simulink model "fw_io_out_hw"  (R2026b)
settings: Solver=VariableStepAuto
undefined symbols (not defined in the file or in its folder): CAN, FD, P, Ts
libraries: stm32blockslib x8, stm32f4xxblockslib x4, simulink x1, stmutilitieslib x1
settings Model: Creator=aomar  LastModifiedBy=aomar

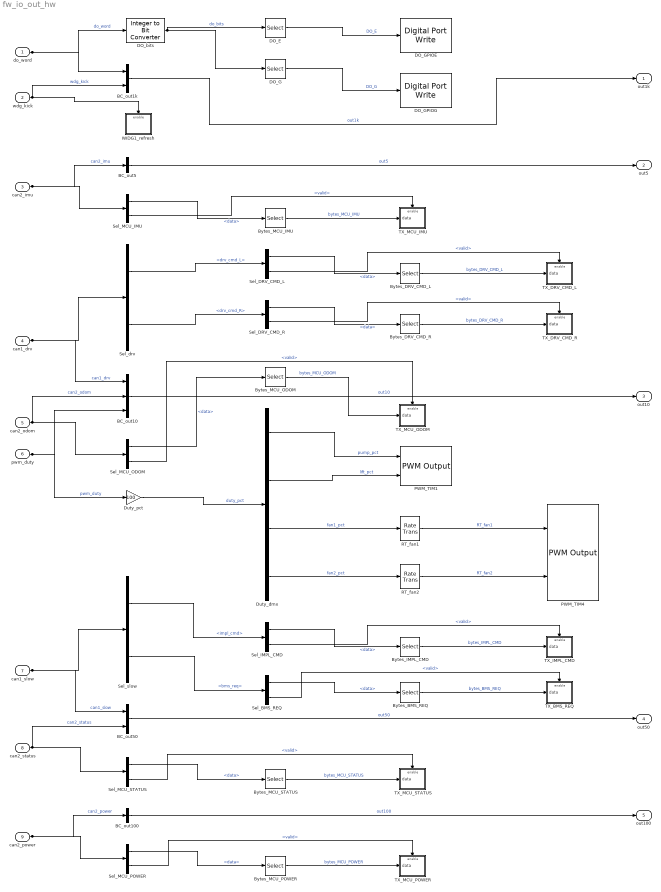
== system fw_io_out_hw ==
  do_word : Inport  OutDataTypeStr=uint32  SampleTime=Ts.base
  wdg_kick : Inport  Port=2  OutDataTypeStr=boolean  SampleTime=Ts.base
  can2_imu : Inport  Port=3  OutDataTypeStr=Bus: Bus_CanFrame64  SampleTime=Ts.imu
  can1_drv : Inport  Port=4  OutDataTypeStr=Bus: Bus_Can1_McuFast  SampleTime=Ts.ctrl
  can2_odom : Inport  Port=5  OutDataTypeStr=Bus: Bus_CanFrame64  SampleTime=Ts.ctrl
  pwm_duty : Inport  Port=6  OutDataTypeStr=single  PortDimensions=4  SampleTime=Ts.ctrl
  can1_slow : Inport  Port=7  OutDataTypeStr=Bus: Bus_Can1_McuSlow  SampleTime=Ts.comm
  can2_status : Inport  Port=8  OutDataTypeStr=Bus: Bus_CanFrame64  SampleTime=Ts.comm
  can2_power : Inport  Port=9  OutDataTypeStr=Bus: Bus_CanFrame64  SampleTime=Ts.hk
  BC_out10 : BusCreator  Inputs=3  OutDataTypeStr=Bus: Bus_McuOut10  NonVirtualBus=on
      settings: InheritFromInputs=off
  BC_out100 : BusCreator  Inputs=1  OutDataTypeStr=Bus: Bus_McuOut100  NonVirtualBus=on
      settings: InheritFromInputs=off
  BC_out1k : BusCreator  Inputs=2  OutDataTypeStr=Bus: Bus_McuOut1k  NonVirtualBus=on
      settings: InheritFromInputs=off
  BC_out5 : BusCreator  Inputs=1  OutDataTypeStr=Bus: Bus_McuOut5  NonVirtualBus=on
      settings: InheritFromInputs=off
  BC_out50 : BusCreator  Inputs=2  OutDataTypeStr=Bus: Bus_McuOut50  NonVirtualBus=on
      settings: InheritFromInputs=off
  Bytes_BMS_REQ : Selector  InputPortWidth=8  IndexOptions=Index vector (dialog)  Indices=1:8  OutputSizes=1
  Bytes_DRV_CMD_L : Selector  InputPortWidth=8  IndexOptions=Index vector (dialog)  Indices=1:8  OutputSizes=1
  Bytes_DRV_CMD_R : Selector  InputPortWidth=8  IndexOptions=Index vector (dialog)  Indices=1:8  OutputSizes=1
  Bytes_IMPL_CMD : Selector  InputPortWidth=8  IndexOptions=Index vector (dialog)  Indices=1:8  OutputSizes=1
  Bytes_MCU_IMU : Selector  InputPortWidth=64  IndexOptions=Index vector (dialog)  Indices=1:48  OutputSizes=1
  Bytes_MCU_ODOM : Selector  InputPortWidth=64  IndexOptions=Index vector (dialog)  Indices=1:32  OutputSizes=1
  Bytes_MCU_POWER : Selector  InputPortWidth=64  IndexOptions=Index vector (dialog)  Indices=1:64  OutputSizes=1
  Bytes_MCU_STATUS : Selector  InputPortWidth=64  IndexOptions=Index vector (dialog)  Indices=1:48  OutputSizes=1
  DO_E : Selector  InputPortWidth=32  IndexOptions=Index vector (dialog)  Indices=P.electronics.hw.do_g_pins+(1:P.electronics.hw.do_e_pins)  OutputSizes=1
  DO_G : Selector  InputPortWidth=32  IndexOptions=Index vector (dialog)  Indices=1:P.electronics.hw.do_g_pins  OutputSizes=1
  DO_GPIOE : stm32f4xxblockslib/Digital Port Write  PortName=GPIOE  PinNumber=[0:3]  ReadOperation=off  IOAsArray=on  EnableSimPort=off  hoistedMaskSrc=ECSoC/ECSimCodegen/Digital Port Write
      settings: LibrarySourceBlock=stm32h7xxblockslib/Digital Port Write
  DO_GPIOG : stm32f4xxblockslib/Digital Port Write  PortName=GPIOG  PinNumber=[0:15]  ReadOperation=off  IOAsArray=on  EnableSimPort=off  hoistedMaskSrc=ECSoC/ECSimCodegen/Digital Port Write
      settings: LibrarySourceBlock=stm32h7xxblockslib/Digital Port Write
  DO_bits : simulink/Logic and Bit Operations/Integer to Bit Converter  nbits=32  signedInputValues=Unsigned  bitOrder=LSB first  outDtype=boolean
      settings: LibrarySourceBlock=|
      | commutil2/Integer to Bit
      | Converter
  Duty_dmx : Demux
  Duty_pct : Gain  Gain=100
  IWDG1_refresh : Subsystem
  PWM_TIM1 : stm32f4xxblockslib/PWM Output  ProcessorFamily=STM32G4  TimerModule=TIM1  DutycycleUnits=Percentage  EnableChannel1=on  EnableCaptureCompare1Input=off  EnableCaptureCompare1ComplementaryInput=off  EnableOutputCompare1ModeInput=off  EnableChannel2=on  EnableCaptureCompare2Input=off  EnableCaptureCompare2ComplementaryInput=off  EnableOutputCompare2ModeInput=off  EnableChannel3=off  EnableCaptureCompare3Input=off  EnableCaptureCompare3ComplementaryInput=off  EnableOutputCompare3ModeInput=off  EnableChannel4=off  EnableCaptureCompare4Input=off  EnableCaptureCompare4ComplementaryInput=off  EnableOutputCompare4ModeInput=off  EnableChannel5=off  EnableCaptureCompare5Input=off  EnableOutputCompare5ModeInput=off  EnableChannel6=off  EnableCaptureCompare6Input=off  EnableOutputCompare6ModeInput=off  EnableCounterInput=off  EnableMainOutputInput=off  EnableFrequencyInput=off  SetRCAfterCE=off  OutputDirection=off  OutputMainOutputEnableStatus=off  SampleTime=Ts.ctrl  EnableSimPort=off  EnableUpdateEvent=off  EnableCaptureCompare1Event=off  EnableCaptureCompare2Event=off  EnableCaptureCompare3Event=off  EnableCaptureCompare4Event=off  EnableTriggerEvent=off  EnableBreakEvent=off  EnableBreakEvent2=off  hoistedMaskSrc=ECSoC/ECSimCodegen/PWM Output
      settings: LibrarySourceBlock=stm32h7xxblockslib/PWM Output
  PWM_TIM4 : stm32f4xxblockslib/PWM Output  ProcessorFamily=STM32G4  TimerModule=TIM4  DutycycleUnits=Percentage  EnableChannel1=on  EnableCaptureCompare1Input=off  EnableCaptureCompare1ComplementaryInput=off  EnableOutputCompare1ModeInput=off  EnableChannel2=on  EnableCaptureCompare2Input=off  EnableCaptureCompare2ComplementaryInput=off  EnableOutputCompare2ModeInput=off  EnableChannel3=off  EnableCaptureCompare3Input=off  EnableCaptureCompare3ComplementaryInput=off  EnableOutputCompare3ModeInput=off  EnableChannel4=off  EnableCaptureCompare4Input=off  EnableCaptureCompare4ComplementaryInput=off  EnableOutputCompare4ModeInput=off  EnableChannel5=off  EnableCaptureCompare5Input=off  EnableOutputCompare5ModeInput=off  EnableChannel6=off  EnableCaptureCompare6Input=off  EnableOutputCompare6ModeInput=off  EnableCounterInput=off  EnableMainOutputInput=off  EnableFrequencyInput=off  SetRCAfterCE=off  OutputDirection=off  OutputMainOutputEnableStatus=off  SampleTime=Ts.hk  EnableSimPort=off  EnableUpdateEvent=off  EnableCaptureCompare1Event=off  EnableCaptureCompare2Event=off  EnableCaptureCompare3Event=off  EnableCaptureCompare4Event=off  EnableTriggerEvent=off  EnableBreakEvent=off  EnableBreakEvent2=off  hoistedMaskSrc=ECSoC/ECSimCodegen/PWM Output
      settings: LibrarySourceBlock=stm32h7xxblockslib/PWM Output
  RT_fan1 : RateTransition  OutPortSampleTime=Ts.hk
  RT_fan2 : RateTransition  OutPortSampleTime=Ts.hk
  Sel_BMS_REQ : BusSelector  OutputSignals=data,valid
  Sel_DRV_CMD_L : BusSelector  OutputSignals=data,valid
  Sel_DRV_CMD_R : BusSelector  OutputSignals=data,valid
  Sel_IMPL_CMD : BusSelector  OutputSignals=data,valid
  Sel_MCU_IMU : BusSelector  OutputSignals=data,valid
  Sel_MCU_ODOM : BusSelector  OutputSignals=data,valid
  Sel_MCU_POWER : BusSelector  OutputSignals=data,valid
  Sel_MCU_STATUS : BusSelector  OutputSignals=data,valid
  Sel_drv : BusSelector  OutputSignals=drv_cmd_L,drv_cmd_R
  Sel_slow : BusSelector  OutputSignals=impl_cmd,bms_req
  TX_BMS_REQ : Subsystem
  TX_DRV_CMD_L : Subsystem
  TX_DRV_CMD_R : Subsystem
  TX_IMPL_CMD : Subsystem
  TX_MCU_IMU : Subsystem
  TX_MCU_ODOM : Subsystem
  TX_MCU_POWER : Subsystem
  TX_MCU_STATUS : Subsystem
  out1k : Outport  OutDataTypeStr=Bus: Bus_McuOut1k
  out5 : Outport  Port=2  OutDataTypeStr=Bus: Bus_McuOut5
  out10 : Outport  Port=3  OutDataTypeStr=Bus: Bus_McuOut10
  out50 : Outport  Port=4  OutDataTypeStr=Bus: Bus_McuOut50
  out100 : Outport  Port=5  OutDataTypeStr=Bus: Bus_McuOut100
  wires:
  do_word/1 -> DO_bits/1, BC_out1k/1  "do_word"
  wdg_kick/1 -> IWDG1_refresh/Enable, BC_out1k/2  "wdg_kick"
  can2_imu/1 -> BC_out5/1, Sel_MCU_IMU/1  "can2_imu"
  can1_drv/1 -> Sel_drv/1, BC_out10/1  "can1_drv"
  can2_odom/1 -> Sel_MCU_ODOM/1, BC_out10/2  "can2_odom"
  pwm_duty/1 -> BC_out10/3, Duty_pct/1  "pwm_duty"
  can1_slow/1 -> Sel_slow/1, BC_out50/1  "can1_slow"
  can2_status/1 -> Sel_MCU_STATUS/1, BC_out50/2  "can2_status"
  can2_power/1 -> BC_out100/1, Sel_MCU_POWER/1  "can2_power"
  BC_out1k/1 -> out1k/1  "out1k"
  BC_out5/1 -> out5/1  "out5"
  Sel_MCU_IMU/1 -> Bytes_MCU_IMU/1  "<data>"
  Sel_MCU_IMU/2 -> TX_MCU_IMU/Enable  "<valid>"
  Sel_drv/1 -> Sel_DRV_CMD_L/1  "<drv_cmd_L>"
  Sel_drv/2 -> Sel_DRV_CMD_R/1  "<drv_cmd_R>"
  BC_out10/1 -> out10/1  "out10"
  Sel_MCU_ODOM/1 -> Bytes_MCU_ODOM/1  "<data>"
  Sel_MCU_ODOM/2 -> TX_MCU_ODOM/Enable  "<valid>"
  Sel_slow/1 -> Sel_IMPL_CMD/1  "<impl_cmd>"
  Sel_slow/2 -> Sel_BMS_REQ/1  "<bms_req>"
  BC_out50/1 -> out50/1  "out50"
  Sel_MCU_STATUS/1 -> Bytes_MCU_STATUS/1  "<data>"
  Sel_MCU_STATUS/2 -> TX_MCU_STATUS/Enable  "<valid>"
  BC_out100/1 -> out100/1  "out100"
  Sel_MCU_POWER/1 -> Bytes_MCU_POWER/1  "<data>"
  Sel_MCU_POWER/2 -> TX_MCU_POWER/Enable  "<valid>"
  Duty_pct/1 -> Duty_dmx/1  "duty_pct"
  DO_bits/1 -> DO_G/1, DO_E/1  "do_bits"
  Sel_DRV_CMD_L/1 -> Bytes_DRV_CMD_L/1  "<data>"
  Sel_DRV_CMD_L/2 -> TX_DRV_CMD_L/Enable  "<valid>"
  Sel_DRV_CMD_R/1 -> Bytes_DRV_CMD_R/1  "<data>"
  Sel_DRV_CMD_R/2 -> TX_DRV_CMD_R/Enable  "<valid>"
  Duty_dmx/1 -> PWM_TIM1/1  "pump_pct"
  Duty_dmx/2 -> PWM_TIM1/2  "lift_pct"
  Duty_dmx/3 -> RT_fan1/1  "fan1_pct"
  Duty_dmx/4 -> RT_fan2/1  "fan2_pct"
  Sel_IMPL_CMD/1 -> Bytes_IMPL_CMD/1  "<data>"
  Sel_IMPL_CMD/2 -> TX_IMPL_CMD/Enable  "<valid>"
  Sel_BMS_REQ/1 -> Bytes_BMS_REQ/1  "<data>"
  Sel_BMS_REQ/2 -> TX_BMS_REQ/Enable  "<valid>"
  DO_E/1 -> DO_GPIOE/1  "DO_E"
  DO_G/1 -> DO_GPIOG/1  "DO_G"
  Bytes_MCU_IMU/1 -> TX_MCU_IMU/1(data)  "bytes_MCU_IMU"
  Bytes_MCU_ODOM/1 -> TX_MCU_ODOM/1(data)  "bytes_MCU_ODOM"
  Bytes_MCU_STATUS/1 -> TX_MCU_STATUS/1(data)  "bytes_MCU_STATUS"
  Bytes_MCU_POWER/1 -> TX_MCU_POWER/1(data)  "bytes_MCU_POWER"
  Bytes_DRV_CMD_L/1 -> TX_DRV_CMD_L/1(data)  "bytes_DRV_CMD_L"
  Bytes_DRV_CMD_R/1 -> TX_DRV_CMD_R/1(data)  "bytes_DRV_CMD_R"
  RT_fan1/1 -> PWM_TIM4/1  "RT_fan1"
  RT_fan2/1 -> PWM_TIM4/2  "RT_fan2"
  Bytes_IMPL_CMD/1 -> TX_IMPL_CMD/1(data)  "bytes_IMPL_CMD"
  Bytes_BMS_REQ/1 -> TX_BMS_REQ/1(data)  "bytes_BMS_REQ"

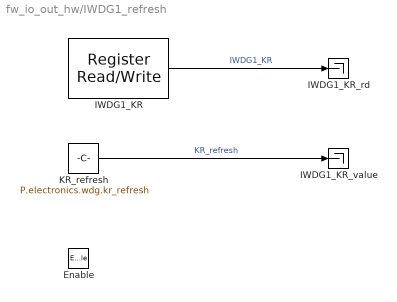
== system fw_io_out_hw/IWDG1_refresh ==
  Enable : EnablePort
  IWDG1_KR : stmutilitieslib/Register Read//Write  Description=INTENDED (set in the T17 board setup): tgtHW 'STM32H7xx Based', devID 'STM32H743', regGrpName 'IWDG1', regName 'KR', opCode 'Write'.  tgtHW=STM32F4xx Based  devID=STM32F401  regGrpName=ADC_Common  regName=CSR  accessMode=Specified bits  opCode=Read  bitsToBeProcessed={ [ 15, 0 ] }  bitFields={'on','All';'off','OVR3';'off','STRT3';'off','JSTRT3';'off','JEOC3';'off','EOC3';'off','AWD3';'off','OVR2';'off','STRT2';'off','JSTRT2';'off','JEOC2';'off','EOC2';'off','AWD2';'off','OVR1';'off','STRT1';'off','JSTRT1';'off','JEOC1';'off','EOC1';'off','AWD1'}  SampleTime=1
  IWDG1_KR_rd : Terminator
  IWDG1_KR_value : Terminator
  KR_refresh : Constant  Value=P.electronics.wdg.kr_refresh  OutDataTypeStr=uint32  SampleTime=-1
  wires:
  KR_refresh/1 -> IWDG1_KR_value/1  "KR_refresh"
  IWDG1_KR/1 -> IWDG1_KR_rd/1  "IWDG1_KR"

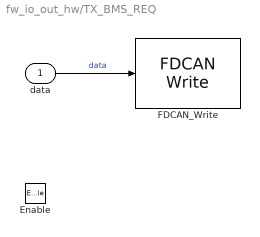
== system fw_io_out_hw/TX_BMS_REQ ==
  data : Inport
  Enable : EnablePort
  FDCAN_Write : stm32blockslib/FDCAN Write  FDCANModule=FDCAN1  BlockMode=Transmit  OperationReadMode=Data  OperationWriteMode=Data  ReadSource=FIFO 0  BufferNumber=0  OutputTypeReadMode=Unpacked  DataFormatWriteMode=Raw data  CANFrameType=CAN  IdentifierTypeVia=Dialog  IdentifierType=Standard (11-bit identifier)  IdentifierVia=Dialog  Identifier=P.electronics.can.id.bms_req  DataLengthVia=Dialog  DataLength=8  OutputIdType=off  IsBitRateSwitchingEnabled=off  TransmitRemoteFrame=off  OutputFrameType=off  OutputBRS=off  OutputRemoteFrame=off  OutputTxFifoLevel=off  OutputRxFifoLevel=off  OutputStatus=off  Timeout=0.001  SampleTime=-1
      settings: LibrarySourceBlock=stm32h7xxblockslib/FDCAN Write
  wires:
  data/1 -> FDCAN_Write/1  "data"

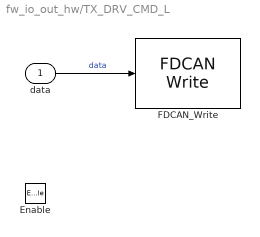
== system fw_io_out_hw/TX_DRV_CMD_L ==
  data : Inport
  Enable : EnablePort
  FDCAN_Write : stm32blockslib/FDCAN Write  FDCANModule=FDCAN1  BlockMode=Transmit  OperationReadMode=Data  OperationWriteMode=Data  ReadSource=FIFO 0  BufferNumber=0  OutputTypeReadMode=Unpacked  DataFormatWriteMode=Raw data  CANFrameType=CAN  IdentifierTypeVia=Dialog  IdentifierType=Standard (11-bit identifier)  IdentifierVia=Dialog  Identifier=P.drive.can.id_cmd+1  DataLengthVia=Dialog  DataLength=8  OutputIdType=off  IsBitRateSwitchingEnabled=off  TransmitRemoteFrame=off  OutputFrameType=off  OutputBRS=off  OutputRemoteFrame=off  OutputTxFifoLevel=off  OutputRxFifoLevel=off  OutputStatus=off  Timeout=0.001  SampleTime=-1
      settings: LibrarySourceBlock=stm32h7xxblockslib/FDCAN Write
  wires:
  data/1 -> FDCAN_Write/1  "data"

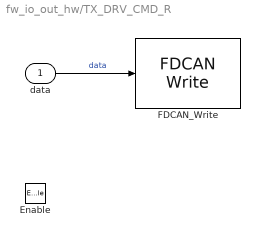
== system fw_io_out_hw/TX_DRV_CMD_R ==
  data : Inport
  Enable : EnablePort
  FDCAN_Write : stm32blockslib/FDCAN Write  FDCANModule=FDCAN1  BlockMode=Transmit  OperationReadMode=Data  OperationWriteMode=Data  ReadSource=FIFO 0  BufferNumber=0  OutputTypeReadMode=Unpacked  DataFormatWriteMode=Raw data  CANFrameType=CAN  IdentifierTypeVia=Dialog  IdentifierType=Standard (11-bit identifier)  IdentifierVia=Dialog  Identifier=P.drive.can.id_cmd+2  DataLengthVia=Dialog  DataLength=8  OutputIdType=off  IsBitRateSwitchingEnabled=off  TransmitRemoteFrame=off  OutputFrameType=off  OutputBRS=off  OutputRemoteFrame=off  OutputTxFifoLevel=off  OutputRxFifoLevel=off  OutputStatus=off  Timeout=0.001  SampleTime=-1
      settings: LibrarySourceBlock=stm32h7xxblockslib/FDCAN Write
  wires:
  data/1 -> FDCAN_Write/1  "data"

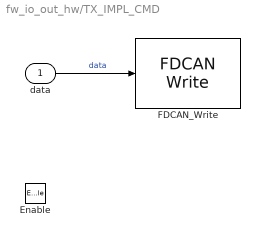
== system fw_io_out_hw/TX_IMPL_CMD ==
  data : Inport
  Enable : EnablePort
  FDCAN_Write : stm32blockslib/FDCAN Write  FDCANModule=FDCAN1  BlockMode=Transmit  OperationReadMode=Data  OperationWriteMode=Data  ReadSource=FIFO 0  BufferNumber=0  OutputTypeReadMode=Unpacked  DataFormatWriteMode=Raw data  CANFrameType=CAN  IdentifierTypeVia=Dialog  IdentifierType=Standard (11-bit identifier)  IdentifierVia=Dialog  Identifier=P.electronics.can.id.impl_cmd  DataLengthVia=Dialog  DataLength=8  OutputIdType=off  IsBitRateSwitchingEnabled=off  TransmitRemoteFrame=off  OutputFrameType=off  OutputBRS=off  OutputRemoteFrame=off  OutputTxFifoLevel=off  OutputRxFifoLevel=off  OutputStatus=off  Timeout=0.001  SampleTime=-1
      settings: LibrarySourceBlock=stm32h7xxblockslib/FDCAN Write
  wires:
  data/1 -> FDCAN_Write/1  "data"

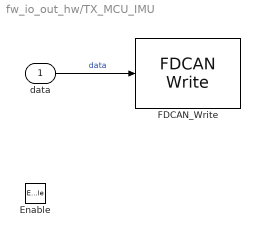
== system fw_io_out_hw/TX_MCU_IMU ==
  data : Inport
  Enable : EnablePort
  FDCAN_Write : stm32blockslib/FDCAN Write  FDCANModule=FDCAN2  BlockMode=Transmit  OperationReadMode=Data  OperationWriteMode=Data  ReadSource=FIFO 0  BufferNumber=0  OutputTypeReadMode=Unpacked  DataFormatWriteMode=Raw data  CANFrameType=CAN-FD  IdentifierTypeVia=Dialog  IdentifierType=Standard (11-bit identifier)  IdentifierVia=Dialog  Identifier=P.electronics.can.id.mcu_imu  DataLengthVia=Dialog  DataLength=48  OutputIdType=off  IsBitRateSwitchingEnabled=on  TransmitRemoteFrame=off  OutputFrameType=off  OutputBRS=off  OutputRemoteFrame=off  OutputTxFifoLevel=off  OutputRxFifoLevel=off  OutputStatus=off  Timeout=0.001  SampleTime=-1
      settings: LibrarySourceBlock=stm32h7xxblockslib/FDCAN Write
  wires:
  data/1 -> FDCAN_Write/1  "data"

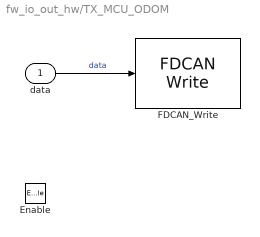
== system fw_io_out_hw/TX_MCU_ODOM ==
  data : Inport
  Enable : EnablePort
  FDCAN_Write : stm32blockslib/FDCAN Write  FDCANModule=FDCAN2  BlockMode=Transmit  OperationReadMode=Data  OperationWriteMode=Data  ReadSource=FIFO 0  BufferNumber=0  OutputTypeReadMode=Unpacked  DataFormatWriteMode=Raw data  CANFrameType=CAN-FD  IdentifierTypeVia=Dialog  IdentifierType=Standard (11-bit identifier)  IdentifierVia=Dialog  Identifier=P.electronics.can.id.mcu_odom  DataLengthVia=Dialog  DataLength=32  OutputIdType=off  IsBitRateSwitchingEnabled=on  TransmitRemoteFrame=off  OutputFrameType=off  OutputBRS=off  OutputRemoteFrame=off  OutputTxFifoLevel=off  OutputRxFifoLevel=off  OutputStatus=off  Timeout=0.001  SampleTime=-1
      settings: LibrarySourceBlock=stm32h7xxblockslib/FDCAN Write
  wires:
  data/1 -> FDCAN_Write/1  "data"

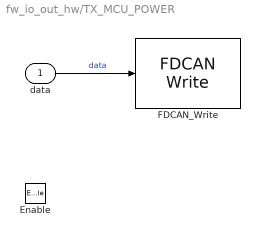
== system fw_io_out_hw/TX_MCU_POWER ==
  data : Inport
  Enable : EnablePort
  FDCAN_Write : stm32blockslib/FDCAN Write  FDCANModule=FDCAN2  BlockMode=Transmit  OperationReadMode=Data  OperationWriteMode=Data  ReadSource=FIFO 0  BufferNumber=0  OutputTypeReadMode=Unpacked  DataFormatWriteMode=Raw data  CANFrameType=CAN-FD  IdentifierTypeVia=Dialog  IdentifierType=Standard (11-bit identifier)  IdentifierVia=Dialog  Identifier=P.electronics.can.id.mcu_power  DataLengthVia=Dialog  DataLength=64  OutputIdType=off  IsBitRateSwitchingEnabled=on  TransmitRemoteFrame=off  OutputFrameType=off  OutputBRS=off  OutputRemoteFrame=off  OutputTxFifoLevel=off  OutputRxFifoLevel=off  OutputStatus=off  Timeout=0.001  SampleTime=-1
      settings: LibrarySourceBlock=stm32h7xxblockslib/FDCAN Write
  wires:
  data/1 -> FDCAN_Write/1  "data"

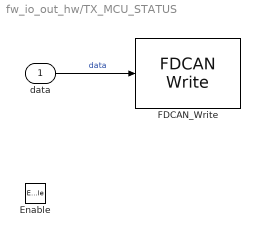
== system fw_io_out_hw/TX_MCU_STATUS ==
  data : Inport
  Enable : EnablePort
  FDCAN_Write : stm32blockslib/FDCAN Write  FDCANModule=FDCAN2  BlockMode=Transmit  OperationReadMode=Data  OperationWriteMode=Data  ReadSource=FIFO 0  BufferNumber=0  OutputTypeReadMode=Unpacked  DataFormatWriteMode=Raw data  CANFrameType=CAN-FD  IdentifierTypeVia=Dialog  IdentifierType=Standard (11-bit identifier)  IdentifierVia=Dialog  Identifier=P.electronics.can.id.mcu_status  DataLengthVia=Dialog  DataLength=48  OutputIdType=off  IsBitRateSwitchingEnabled=on  TransmitRemoteFrame=off  OutputFrameType=off  OutputBRS=off  OutputRemoteFrame=off  OutputTxFifoLevel=off  OutputRxFifoLevel=off  OutputStatus=off  Timeout=0.001  SampleTime=-1
      settings: LibrarySourceBlock=stm32h7xxblockslib/FDCAN Write
  wires:
  data/1 -> FDCAN_Write/1  "data"
